simulink model "KSimulator_kuka_iiwa7_kinCtrl"  (R2021a)
settings: Solver=ode1  StartTime=0.0  StopTime=6  FixedStep=0.001  RelTol=1e-3  EnableMultiTasking=on
undefined symbols (not defined in the file or in its folder): kinematicCtrlOp, plotRobot_KinCtrl, trajGen_abbIRB4Op
CloseFcn:
  | EraseHandles
settings Model: Creator=E. Dean  LastModifiedBy=little_long
settings SolverCC: AlgebraicLoopSolver=TrustRegion
settings DataIOCC: LimitDataPoints=on  SaveFormat=Array  SignalLoggingSaveFormat=ModelDataLogs  ReturnWorkspaceOutputs=off
settings OptimizationCC: ExpressionDepthLimit=2147483647  LifeSpan=inf
settings DebuggingCC: UnderspecifiedInitializationDetection=Classic  MergeDetectMultiDrivingBlocksExec=none  SolverPrmCheckMsg=warning  FcnCallInpInsideContextMsg=warning  AllowSymbolicDim=off  StateNameClashWarn=warning  SFUnexpectedBacktrackingDiag=warning  SFNoUnconditionalDefaultTransitionDiag=warning  SFExecutionAtInitializationDiag=none  SFMachineParentedDataDiag=warning  ArithmeticOperatorsInVariantConditions=warning
settings HardwareCC: ProdBitPerPointer=32  ProdBitPerSizeT=32  ProdBitPerPtrDiffT=32  ProdLargestAtomicFloat=None  ProdIntDivRoundTo=Undefined  ProdEndianess=Unspecified  ProdWordSize=32  ProdHWDeviceType=32-bit Generic
settings ModelReferenceCC: PropagateSignalLabelsOutOfModel=off
settings SFSimCC: SimUseLocalCustomCode=off  CustomCodeUndefinedFunction=UseInterfaceOnly
settings RTWCC: RTWUseLocalCustomCode=off
settings CodeAppCC: StateflowObjectComments=on
settings GRTTargetCC: TargetLangStandard=C89/C90 (ANSI)  CombineOutputUpdateFcns=off  GRTInterface=on
settings ConfigComp: CovMetricSettings=dw  CovSaveCumulativeToWorkspaceVar=on  CovSaveSingleToWorkspaceVar=on  CovExternalEMLEnable=off  CovSFcnEnable=off

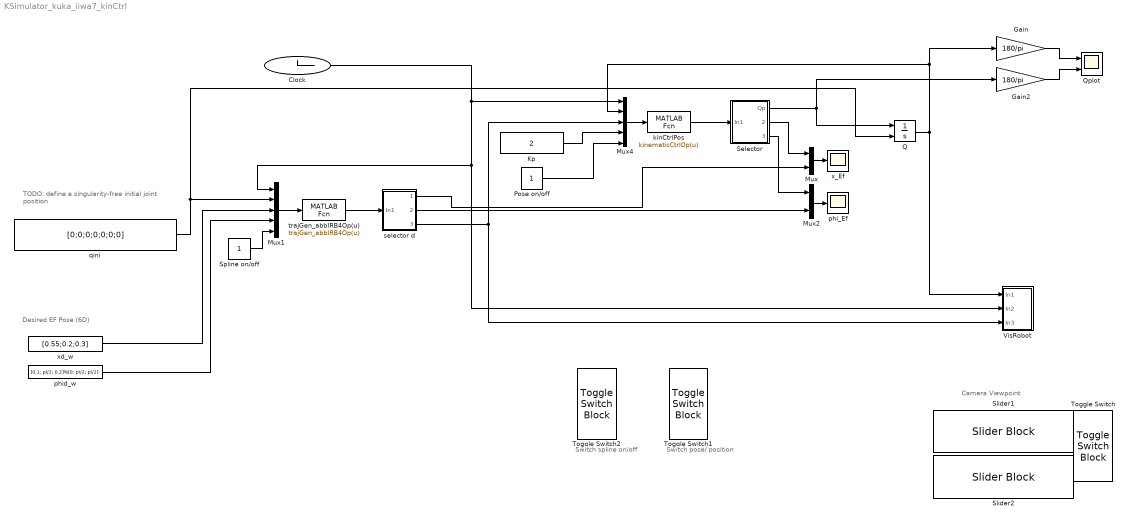
== system KSimulator_kuka_iiwa7_kinCtrl ==
  note: Desired EF Pose (6D)
  note: TODO: define a singularity-free
      | initial joint position
  note: Camera Viewpoint
  note: Switch
      | pose/ position
  note: Switch
      | spline on/off
  Clock : Clock
  Gain : Gain  Gain=180/pi
  Gain2 : Gain  Gain=180/pi
  Kp : Constant  Value=2
  Mux : Mux  Inputs=2
  Mux1 : Mux  Inputs=5
  Mux2 : Mux  Inputs=2
  Mux4 : Mux  Inputs=5
  Pose on/off : Constant
  Q : Integrator  InitialConditionSource=external
  Qplot : Scope  NumInputPorts=2
  Selector : Subsystem
  Slider1 : SliderBlock  ScaleMin=-180  ScaleMax=180  TickInterval=180
  Slider2 : SliderBlock  ScaleMin=-180  ScaleMax=180  TickInterval=180
  Spline on/off : Constant
  Toggle Switch : ToggleSwitchBlock
      settings: Values={{'Off', 'On'}, [0 1]}
  Toggle Switch1 : ToggleSwitchBlock
      settings: Values={{'Off', 'On'}, [0 1]}
  Toggle Switch2 : ToggleSwitchBlock
      settings: Values={{'Off', 'On'}, [0 1]}
  VisRobot : Subsystem
  kinCtrlPos : MATLABFcn  MATLABFcn=kinematicCtrlOp(u)  OutputDimensions=13
  phi_Ef : Scope
  phid_w : Constant  Value=[0.1; pi/2; 0.2]%[0; pi/2; pi/2]
  qini : Constant  Value=[0;0;0;0;0;0;0]
  selector d : Subsystem
  trajGen_abbIRB4Op(u) : MATLABFcn  MATLABFcn=trajGen_abbIRB4Op(u)  OutputDimensions=22
  x_Ef : Scope
  xd_w : Constant  Value=[0.55;0.2;0.3]
  wires:
  Clock/1 -> VisRobot/2(In2), Mux1/1, Mux4/1
  qini/1 -> Mux1/2, Q/2
  Gain/1 -> Qplot/1
  Gain2/1 -> Qplot/2
  Mux4/1 -> kinCtrlPos/1
  Mux1/1 -> trajGen_abbIRB4Op(u)/1
  Kp/1 -> Mux4/4
  Q/1 -> VisRobot/1(In1), Gain/1, Mux4/2
  phid_w/1 -> Mux1/4
  Pose on/off/1 -> Mux4/5
  Selector/1(Qp) -> Q/1, Gain2/1
  kinCtrlPos/1 -> Selector/1(In1)
  Mux/1 -> x_Ef/1
  Mux2/1 -> phi_Ef/1
  Selector/2(xef_0) -> Mux/1
  Selector/3(phief_0) -> Mux2/1
  xd_w/1 -> Mux1/3
  Spline on/off/1 -> Mux1/5
  selector d/3(Hd_w) -> VisRobot/3(In3), Mux4/3
  trajGen_abbIRB4Op(u)/1 -> selector d/1(In1)
  selector d/1(xd_w) -> Mux/2
  selector d/2(phid_w) -> Mux2/2

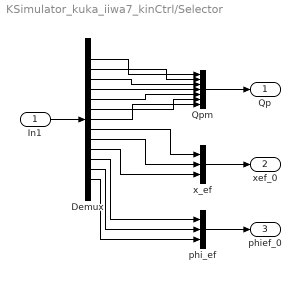
== system KSimulator_kuka_iiwa7_kinCtrl/Selector ==
  In1 : Inport
  Demux : Demux  Outputs=13
  Qpm : Mux  Inputs=7
  phi_ef : Mux  Inputs=3
  x_ef : Mux  Inputs=3
  Qp : Outport
  xef_0 : Outport  Port=2
  phief_0 : Outport  Port=3
  wires:
  In1/1 -> Demux/1
  Demux/8 -> x_ef/1
  Demux/3 -> Qpm/3
  Demux/2 -> Qpm/2
  phi_ef/1 -> phief_0/1
  Demux/4 -> Qpm/4
  x_ef/1 -> xef_0/1
  Demux/7 -> Qpm/7
  Demux/5 -> Qpm/5
  Demux/1 -> Qpm/1
  Demux/11 -> phi_ef/1
  Demux/12 -> phi_ef/2
  Demux/6 -> Qpm/6
  Demux/9 -> x_ef/2
  Demux/13 -> phi_ef/3
  Qpm/1 -> Qp/1
  Demux/10 -> x_ef/3

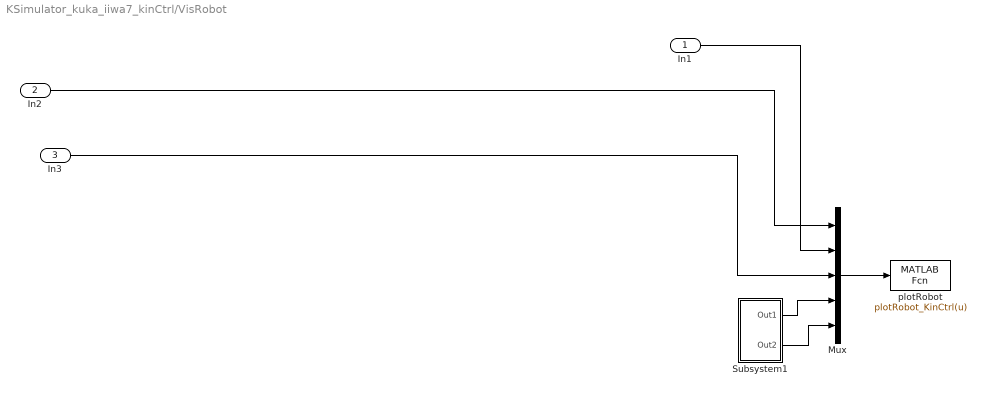
== system KSimulator_kuka_iiwa7_kinCtrl/VisRobot ==
  In1 : Inport
  In2 : Inport  Port=2
  In3 : Inport  Port=3
  Mux : Mux  Inputs=5
  Subsystem1 : Subsystem
  plotRobot : MATLABFcn  MATLABFcn=plotRobot_KinCtrl(u)  OutputDimensions=0
  wires:
  Subsystem1/1(Out1) -> Mux/4
  In2/1 -> Mux/1
  Subsystem1/2(Out2) -> Mux/5
  In3/1 -> Mux/3
  Mux/1 -> plotRobot/1
  In1/1 -> Mux/2

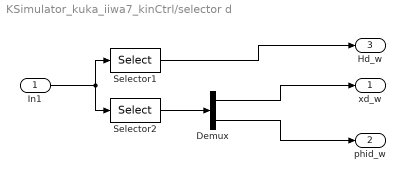
== system KSimulator_kuka_iiwa7_kinCtrl/selector d ==
  In1 : Inport
  Demux : Demux  Outputs=2
  Selector1 : Selector  InputPortWidth=22  IndexOptions=Index vector (dialog)  Indices=[1:16]  OutputSizes=1
  Selector2 : Selector  InputPortWidth=22  IndexOptions=Index vector (dialog)  Indices=[17:22]  OutputSizes=1
  xd_w : Outport
  phid_w : Outport  Port=2
  Hd_w : Outport  Port=3
  wires:
  Demux/2 -> phid_w/1
  Demux/1 -> xd_w/1
  Selector1/1 -> Hd_w/1
  In1/1 -> Selector1/1, Selector2/1
  Selector2/1 -> Demux/1

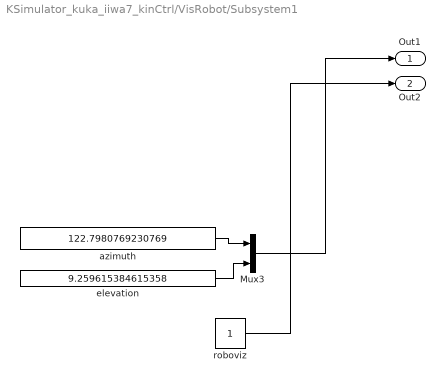
== system KSimulator_kuka_iiwa7_kinCtrl/VisRobot/Subsystem1 ==
  Mux3 : Mux  Inputs=2
  azimuth : Constant  Value=122.7980769230769
  elevation : Constant  Value=9.259615384615358
  roboviz : Constant
  Out1 : Outport
  Out2 : Outport  Port=2
  wires:
  azimuth/1 -> Mux3/1
  roboviz/1 -> Out2/1
  elevation/1 -> Mux3/2
  Mux3/1 -> Out1/1
